simulink model "tdpLearningReplay"  (R2026b)
settings: Solver=FixedStepDiscrete  StopTime=2  FixedStep=P.dt
model workspace (MAT data in the model file):
  P.L = 9
  P.W = 6
  P.goalD = 0.6
  P.goalW = 2.6
  P.goalAreaL = 1
  P.goalAreaW = 3
  P.penMark = 1.5
  P.centreD = 1.5
  P.border = 1
  P.penAreaL = 2
  P.penAreaW = 5
  P.ballR = 0.07
  P.ballDecel = 0.4
  P.ballRestit = 0.5
  P.ballRobotE = 0.3
  P.robotR = 0.15
  P.vFwd = 0.25
  P.vBack = 0.12
  P.vSide = 0.15
  P.wMax = 0.785398163397
  P.Kp = 0.8
  P.Kw = 2
  P.avoidR = 0.7
  P.avoidGain = 0.6
  P.ballAvoidR = 0.35
  P.approachDist = 0.45
  P.kickRange = 0.28
  P.stepInSpeed = 0.1
  P.kickAlign = 0.349065850399
  P.behindTol = 0.523598775598
  P.kickNoise = 0.10471975512
  P.kickCooldown = 1
  P.shotSpeed = 1.8
  P.dribbleSpeed = 0.6
  P.maxKickSpeed = 2.2
  P.roleHyst = 0.4
  P.shootDist = 3
  P.defDist = 1.8
  P.nPerTeam = 4
  P.dt = 0.05
  P.Tmatch = 600
  P.restartPause = 2
  P.outPause = 1
  P.drawEvery = 4
  P.realtime = 0
  P.dirSign = [1 -1]
  P.seed = 1
  P.mode : TdpMode (value not decoded)
  P.rulesProfile : TdpRules (value not decoded)
  P.maxObservationAge = 0.5
  P.walkValidity = 0.1
  P.kickPreparation = 0.2
  P.kickTimeout = 1
  P.recoverTime = 0.5
  P.alignEnter = 0.35
  P.alignExit = 0.45
  P.searchTurnRate = 0.3
  P.fieldOfView = 6.28318530718
  P.observationDelay = 0
  P.observationNoise = 0
  P.fixedStriker = 0
  P.tapSpeed = 0.3
  P.freezeDuringPause = 0
  P.contactIterations = 256
  P.restartOpponentDistance = 0.75
  P.contactTolerance = 1e-10
  scenario : object (value not decoded)
symbols that are objects in the model workspace (value not decoded): scenario
settings Model: DataDictionary=TdpTypes.sldd  Creator=fayne  LastModifiedBy=fayne
settings DataIOCC: SaveOutput=off  SignalLogging=off
settings DebuggingCC: AlgebraicLoopMsg=error

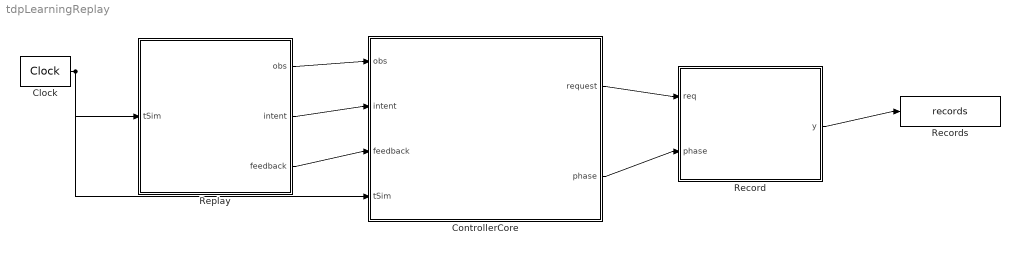
== system tdpLearningReplay ==
  Clock : DigitalClock  SampleTime=P.dt
  ControllerCore : Subsystem
  Record : MATLAB Function  TreatAsAtomicUnit=on
  Records : ToWorkspace  VariableName=records  SampleTime=-1
  Replay : MATLAB Function  TreatAsAtomicUnit=on
  wires:
  Replay/1(obs) -> ControllerCore/1(obs)
  Replay/2(intent) -> ControllerCore/2(intent)
  Replay/3(feedback) -> ControllerCore/3(feedback)
  Clock/1 -> Replay/1(tSim), ControllerCore/4(tSim)
  ControllerCore/1(request) -> Record/1(req)
  ControllerCore/2(phase) -> Record/2(phase)
  Record/1(y) -> Records/1

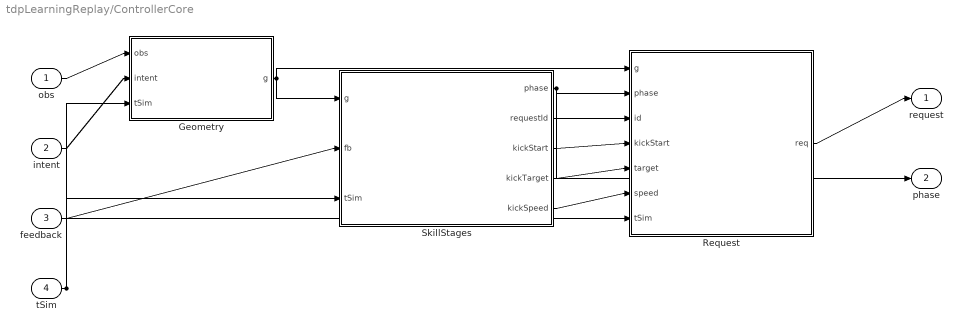
== system tdpLearningReplay/ControllerCore ==
  obs : Inport
  intent : Inport  Port=2
  feedback : Inport  Port=3
  tSim : Inport  Port=4
  Geometry : MATLAB Function  TreatAsAtomicUnit=on
  Request : MATLAB Function  TreatAsAtomicUnit=on
  SkillStages : Stateflow chart  TreatAsAtomicUnit=on
  request : Outport
  phase : Outport  Port=2
  wires:
  Request/1(req) -> request/1
  SkillStages/5(kickSpeed) -> Request/6(speed)
  SkillStages/4(kickTarget) -> Request/5(target)
  SkillStages/3(kickStart) -> Request/4(kickStart)
  SkillStages/2(requestId) -> Request/3(id)
  SkillStages/1(phase) -> phase/1, Request/2(phase)
  feedback/1 -> SkillStages/2(fb)
  Geometry/1(g) -> Request/1(g), SkillStages/1(g)
  tSim/1 -> Request/7(tSim), SkillStages/3(tSim), Geometry/3(tSim)
  intent/1 -> Geometry/2(intent)
  obs/1 -> Geometry/1(obs)

== matlab function tdpLearningReplay/Record ==
  data: req input Bus: RequestBus; y output; phase input Enum: TdpPhase
function y=f(req,phase)
y=[double(req.kind) double(req.requestId) double(phase) req.velocity req.target req.speed req.stamp req.validUntil];
end

== matlab function tdpLearningReplay/Replay ==
  data: tSim input; obs output Bus: ObservationBus; intent output Bus: IntentBus; feedback output Bus: FeedbackBus; scenario parameter; P parameter
function [obs,intent,feedback]=f(tSim,scenario, P)
k=min(numel(scenario),max(1,round(tSim/P.dt)+1));
obs=scenario(k).obs;intent=scenario(k).intent;feedback=scenario(k).feedback;
end

== matlab function tdpLearningReplay/ControllerCore/Geometry ==
  data: obs input Bus: ObservationBus; g output Bus: GeometryBus; intent input Bus: IntentBus; tSim input; P parameter
function g=f(obs,intent,tSim,P)
g=CoreGeometry(obs,intent,tSim,P);
end

== matlab function tdpLearningReplay/ControllerCore/Request ==
  data: g input Bus: GeometryBus; req output Bus: RequestBus; phase input Enum: TdpPhase; id input uint32; kickStart input; target input; speed input; tSim input; P parameter
function req=f(g,phase,id,kickStart,target,speed,tSim,P)
req=EmitRequest(g,phase,id,kickStart,target,speed,tSim,P);
end

== stateflow chart tdpLearningReplay/ControllerCore/SkillStages ==
  settings: updateMethod=DISCRETE  sampleTime=P.dt
  state Idle
    en,du:
    phase=TdpPhase.Idle;
    requestId=requestId+uint32(1);
  state Active
    en,du:
    if P.mode==TdpMode.Compat || phase~=TdpPhase.Kick
    requestId=requestId+uint32(1);
    end
    state Search
      en: phase=TdpPhase.Search;
    state Approach
      en: phase=TdpPhase.Approach;
    state Align
      en: phase=TdpPhase.Align;
    state Kick
      en:
      phase=TdpPhase.Kick;
      requestId=requestId+uint32(1);
      kickStart=tSim;
      kickTarget=g.target;
      kickSpeed=g.speed;
    state Recover
      en:
      phase=TdpPhase.Recover;
      recoverStart=tSim;
    (default) -> Search
    Align -> Kick [order 3] : [g.ready]
    Align -> Search [order 1] : [~g.ballVisible]
    Approach -> Search [order 1] : [~g.ballVisible && g.intent~=TdpAction.Goto]
    Recover -> Search : [tSim-recoverStart>=P.recoverTime]
    Search -> Approach : [g.ballVisible || g.intent==TdpAction.Goto]
    Align -> Approach [order 2] : [g.distance>P.alignExit || g.intent==TdpAction.Goto]
    Approach -> Align [order 2] : [g.distance<P.alignEnter && g.intent~=TdpAction.Goto]
    Kick -> Recover [order 1] : [fb.requestId==requestId && (fb.status==TdpStatus.Done || fb.status==TdpStatus.Failed || fb.status==TdpStatus.Rejected)]
    Kick -> Recover [order 2] : [tSim-kickStart>=P.kickTimeout]
    Kick -> Recover [order 3] : [~g.ballVisible]
  (default) -> Idle : {requestId=uint32(0);kickStart=0;kickTarget=[0 0];kickSpeed=0;recoverStart=0;}
  Active -> Idle : [~g.safe || (~g.running && P.mode==TdpMode.Delayed)]
  Idle -> Active : [g.safe && (g.running || P.mode==TdpMode.Compat)]
  data: g input Bus: GeometryBus size=1; fb input Bus: FeedbackBus size=1; tSim input double size=1; P parameter size=1; phase output Enum: TdpPhase size=1; requestId output uint32 size=1; kickStart output double size=1; kickTarget output double size=[1 2]; kickSpeed output double size=1; recoverStart local double size=1
